simulink model "sf_mealy_traffic_light"  (R2025b)
settings: Solver=FixedStepDiscrete  StartTime=0.0  StopTime=150  FixedStep=.1  RelTol=1e-3  EnableMultiTasking=on
undefined symbols (not defined in the file): DiscIntNeverNeededParam
libraries: simulink x1
settings Model: Creator=The MathWorks, Inc.  LastModifiedBy=The MathWorks, Inc.
settings SolverCC: AlgebraicLoopSolver=TrustRegion
settings DataIOCC: LimitDataPoints=on  SaveFormat=Array  ReturnWorkspaceOutputs=off
settings OptimizationCC: ReuseModelBlockBuffer=off  ExpressionDepthLimit=2147483647.0  InitFltsAndDblsToZero=on  EfficientMapNaN2IntZero=off  LifeSpan=inf
settings DebuggingCC: SaveWithParameterizedLinksMsg=none  UnderspecifiedInitializationDetection=Classic  MergeDetectMultiDrivingBlocksExec=none  SignalResolutionControl=TryResolveAllWithWarning  SolverPrmCheckMsg=warning  MultiTaskDSMMsg=warning  MultiTaskCondExecSysMsg=none  FcnCallInpInsideContextMsg=warning  UnconnectedInputMsg=warning  UnconnectedOutputMsg=warning  UnconnectedLineMsg=warning  StateNameClashWarn=warning  SFUnexpectedBacktrackingDiag=warning  SFNoUnconditionalDefaultTransitionDiag=warning  SFExecutionAtInitializationDiag=none  ArithmeticOperatorsInVariantConditions=warning
settings HardwareCC: ProdBitPerPointer=32.0  ProdBitPerSizeT=32.0  ProdBitPerPtrDiffT=32.0  ProdLargestAtomicFloat=None  ProdIntDivRoundTo=Undefined  ProdEndianess=Unspecified  ProdWordSize=32.0  ProdHWDeviceType=32-bit Generic
settings ModelReferenceCC: EnableRefExpFcnMdlSchedulingChecks=on  PropagateSignalLabelsOutOfModel=off
settings SFSimCC: SimUseLocalCustomCode=off  SimParseCustomCode=off  CustomCodeUndefinedFunction=UseInterfaceOnly
settings RTWCC: RTWUseLocalCustomCode=off  GPUComputeCapability=3.5
settings CodeAppCC: StateflowObjectComments=on
settings GRTTargetCC: TargetFcnLib=ansi_tfl_tmw.mat  TargetLangStandard=C89/C90 (ANSI)  CombineOutputUpdateFcns=off  GRTInterface=on
settings ConfigComp: CovMetricSettings=dw  CovSaveCumulativeToWorkspaceVar=on  CovSaveSingleToWorkspaceVar=on  CovExternalEMLEnable=off  CovSFcnEnable=off

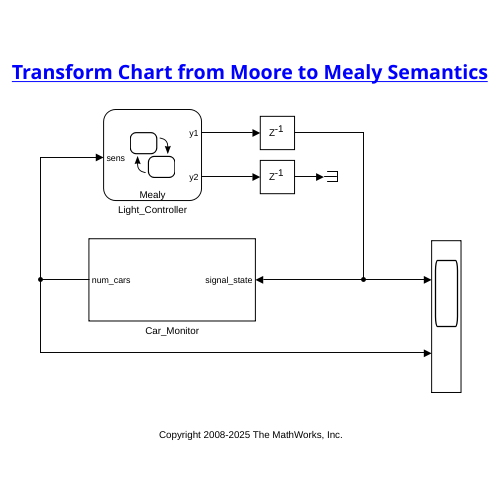
[thumbnail: Simulink's stored preview of the top-level diagram]
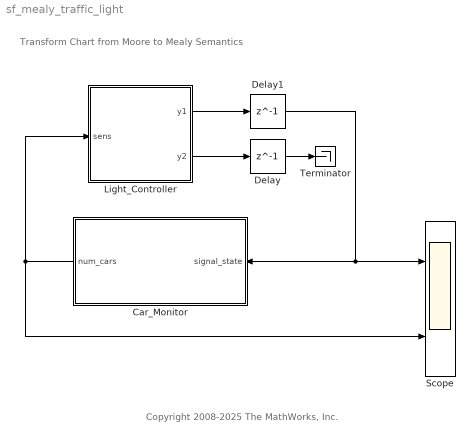
== system sf_mealy_traffic_light ==
  note: Copyright 2008-2025 The MathWorks, Inc.
  note: Transform Chart from Moore to Mealy Semantics
  Car_Monitor : Subsystem
  Delay : Delay  DelayLength=1
  Delay1 : Delay  DelayLength=1
  Light_Controller : Stateflow chart  TreatAsAtomicUnit=on
  Scope : Scope  NumInputPorts=2
      settings: Title=Traffic Light1  ActiveDisplayYMinimum=0.75  ActiveDisplayYMaximum=3.25
  Terminator : Terminator
  wires:
  Car_Monitor/1(num_cars) -> Scope/2, Light_Controller/1(sens)
  Light_Controller/2(y2) -> Delay/1
  Light_Controller/1(y1) -> Delay1/1
  Delay/1 -> Terminator/1
  Delay1/1 -> Scope/1, Car_Monitor/1(signal_state)

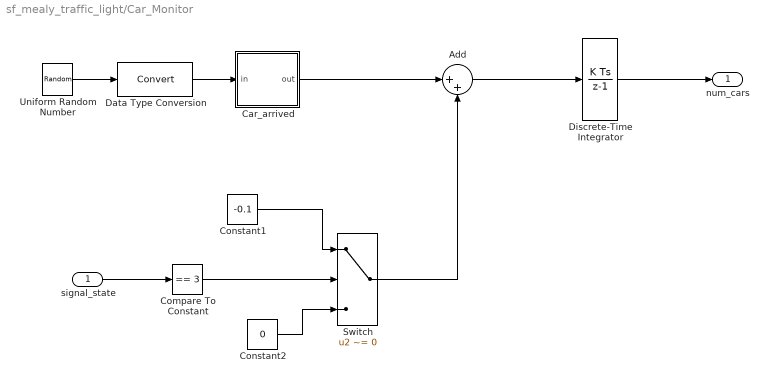
== system sf_mealy_traffic_light/Car_Monitor ==
  signal_state : Inport
  Add : Sum  Inputs=|++
  Car_arrived : Stateflow chart  TreatAsAtomicUnit=on
  Compare To Constant : simulink/Logic and Bit Operations/Compare To Constant  relop===  const=3  OutDataTypeStr=boolean  ZeroCross=off
  Constant1 : Constant  Value=-0.1
  Constant2 : Constant  Value=0
  Data Type Conversion : DataTypeConversion  SaturateOnIntegerOverflow=off  RndMeth=Floor
  Discrete-Time Integrator : DiscreteIntegrator  SampleTime=-1  LimitOutput=on  LowerSaturationLimit=0  ICPrevOutput=DiscIntNeverNeededParam  ICPrevScaledInput=DiscIntNeverNeededParam
  Switch : Switch  Criteria=u2 ~= 0  SaturateOnIntegerOverflow=off  InputSameDT=off
  Uniform Random Number : UniformRandomNumber  Minimum=0  Maximum=100  Seed=177836  SampleTime=0
  num_cars : Outport  VectorParamsAs1DForOutWhenUnconnected=off
  wires:
  Constant1/1 -> Switch/1
  Constant2/1 -> Switch/3
  Discrete-Time Integrator/1 -> num_cars/1
  signal_state/1 -> Compare To Constant/1
  Compare To Constant/1 -> Switch/2
  Switch/1 -> Add/2
  Add/1 -> Discrete-Time Integrator/1
  Car_arrived/1(out) -> Add/1
  Data Type Conversion/1 -> Car_arrived/1(in)
  Uniform Random Number/1 -> Data Type Conversion/1

== stateflow chart sf_mealy_traffic_light/Light_Controller ==
  settings: stateMachineType=MEALY_MACHINE  executeAtInitialization=1
  state Stop
  state StopForTraffic
  state StopToGo
  state GoToStop
  state Go
  (default) -> Stop : {y1 = RED;y2 = GREEN;}
  Stop -> StopForTraffic : after(20,tick)
  StopForTraffic -> StopToGo : [sens]{y1 = RED;y2 = YELLOW;}
  GoToStop -> Stop : after(3,tick){y1 = RED;y2 = GREEN;}
  StopToGo -> Go : after(3,tick){y1 = GREEN;y2 = RED;}
  Go -> GoToStop : after(10,tick){y1 = YELLOW;y2 = RED;}
  data: sens input double; y1 output double; RED constant uint8 =1; YELLOW constant double =2; GREEN constant double =3; y2 output double

== stateflow chart sf_mealy_traffic_light/Car_Monitor/Car_arrived ==
  (default) -> (junction 2) : {out = in > 98;}
  data: in input int8; out output double
